simulink model "ecu_egrg"  (R2026a)
settings: Solver=FixedStepDiscrete  StopTime=10  FixedStep=0.001  SampleTimeConstraint=STIndependent
Description:
  | EGR stall guard. Source of truth for firmware/gen/ecu_egrg.
settings Model: Creator=jj1001000  LastModifiedBy=jj1001000
settings OptimizationCC: DefaultUnderspecifiedDataType=single
settings DebuggingCC: ParameterPrecisionLossMsg=none
settings HardwareCC: ProdLargestAtomicInteger=Long  ProdLargestAtomicFloat=Double  ProdHWDeviceType=ARM Compatible->ARM Cortex-M
settings RTWCC: SystemTargetFile=ert.tlc  GenCodeOnly=on  Description=Embedded Coder
settings ERTTargetCC: UtilityFuncGeneration=Shared location  IncludeMdlTerminateFcn=off  CodeInterfacePackaging=Reusable function  SupportNonFinite=off

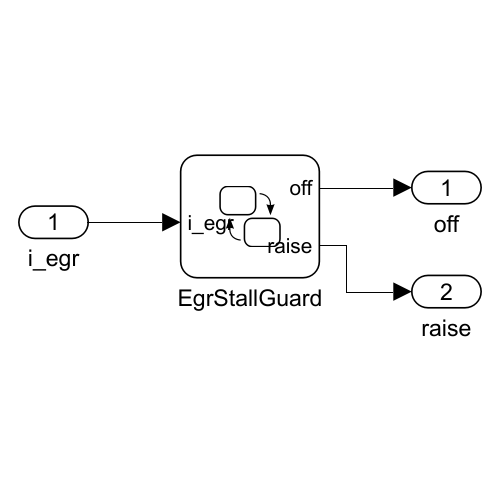
[thumbnail: Simulink's stored preview of the top-level diagram]
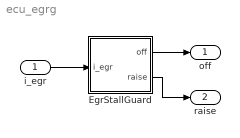
== system ecu_egrg ==
  i_egr : Inport  OutDataTypeStr=single
  EgrStallGuard : Stateflow chart  TreatAsAtomicUnit=on
  off : Outport  OutDataTypeStr=uint8
  raise : Outport  Port=2  OutDataTypeStr=uint8
  wires:
  i_egr/1 -> EgrStallGuard/1(i_egr)
  EgrStallGuard/1(off) -> off/1
  EgrStallGuard/2(raise) -> raise/1

== stateflow chart ecu_egrg/EgrStallGuard ==
  settings: updateMethod=DISCRETE  executeAtInitialization=1
  state Guard
    entry: hot = uint16(0); cool = uint16(0); stalls = uint8(0); raise = uint8(0);
    during: raise = uint8(0);
    if i_egr > single(5)
    hot = min(hot + 1, uint16(1500));
    elseif hot > 0
    hot = hot - 1;
    end
    state NORMAL
      entry: off = uint8(0);
    state COAST
      entry: off = uint8(1);
      during: cool = cool - 1;
    state LOCKED
      entry: off = uint8(1);
    NORMAL -> LOCKED [order 1] : [hot >= uint16(1500) && stalls + 1 >= uint8(3)]{hot = uint16(0); cool = uint16(5000); raise = uint8(1); stalls = uint8(3);}
    (default) -> NORMAL
    NORMAL -> COAST [order 2] : [hot >= uint16(1500)]{hot = uint16(0); cool = uint16(5000); raise = uint8(1); stalls = stalls + 1;}
    COAST -> NORMAL : [cool <= 1]{cool = uint16(0);}
  (default) -> Guard
  data: i_egr input single; off output uint8; raise output uint8; hot local uint16; cool local uint16; stalls local uint8
